simulink model "sschdlexFlybackConverterModel"  (R2026a)
settings: Solver=FixedStepDiscrete  StopTime=200e-6
InitFcn:
  | ts = 2e-008;
libraries: fl_lib x13, nesl_utility x7, ee_lib x2, simulink x1, hdlsllib x1
CloseFcn:
  | clear ts;
settings Model: DataTypeOverride=Off  Creator=The MathWorks, Inc.  LastModifiedBy=The MathWorks, Inc.
settings OptimizationCC: ConditionallyExecuteInputs=off
settings DebuggingCC: AlgebraicLoopMsg=error  SingleTaskRateTransMsg=error  ParameterPrecisionLossMsg=none
settings HardwareCC: ProdHWDeviceType=ASIC/FPGA->ASIC/FPGA  TargetBitPerLong=64.0  TargetBitPerPointer=64.0  TargetBitPerSizeT=64.0  TargetBitPerPtrDiffT=64.0  TargetLongLongMode=on  TargetIntDivRoundTo=Zero  TargetEndianess=LittleEndian  TargetWordSize=64.0  TargetHWDeviceType=Custom Processor->MATLAB Host Computer  ProdEqTarget=off
settings SimscapeCC: SimscapeNominalValues="[{\"value\":\"1\",\"unit\":\"A\"},{\"value\":\"1\",\"unit\":\"bar\"},{\"value\":\"1\",\"unit\":\"cm^2\"},{\"value\":\"1\",\"unit\":\"cm^3/s\"},{\"value\":\"1\",\"unit\":\"kJ/kg\"},{\"value\":\"1\",\"unit\":\"kW\"},{\"value\":\"1\",\"unit\":\"l\"},{\"value\":\"1\",\"unit\":\"N\"},{\"value\":\"1\",\"unit\":\"N*m\"},{\"value\":\"1\",\"unit\":\"V\"}]"  SimscapeLogType=none  SimscapeLogDataHistory=5000.0

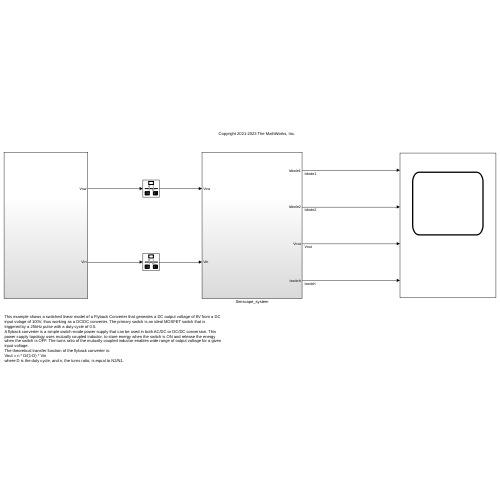
[thumbnail: Simulink's stored preview of the top-level diagram]
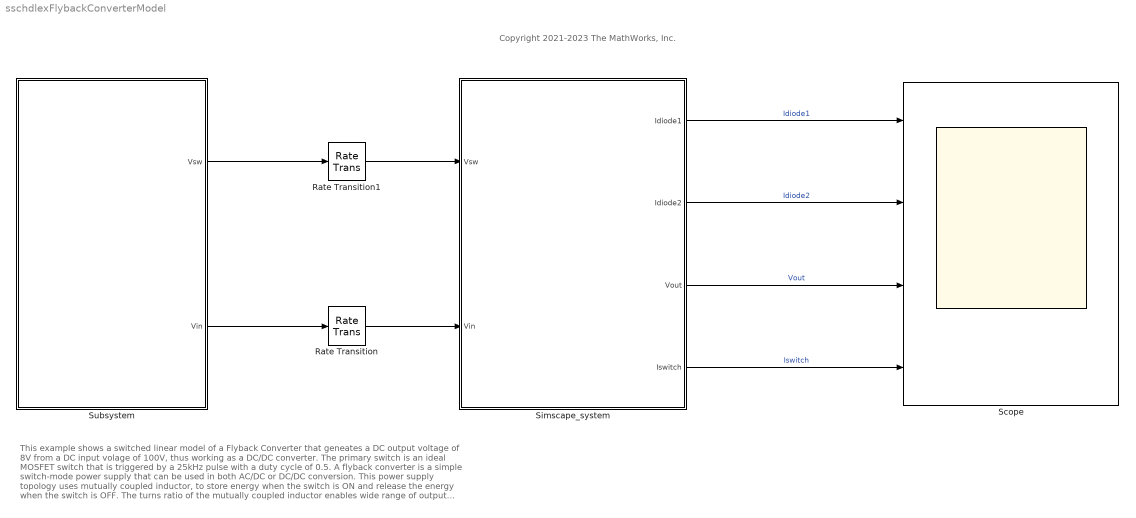
== system sschdlexFlybackConverterModel ==
  note: This example shows a switched linear model of a Flyback Converter that geneates a DC output voltage of 8V from a DC input volage of 100V, thus working as a DC/DC converter. The primary switch is an ideal MOSFET switch that is triggered by a 25kHz pulse with a duty cycle of 0.5.
      | A flyback converter is a simple switch-mode power supply that can be used in both AC/DC or DC/DC conversion. This power supply topology uses mutually coupled inductor, to store energy when the switch is ON and release the energy when the switch is OFF. The turns ratio of the mutually coupled inductor enables wide range of output voltage for a given input voltage.
      | The theoretical transfer function of the flyback converter is:
      | Vout = n * D/(1-D) * Vin
      | where D is the duty cycle, and n, the turns ratio, is equal to N2/N1.
  note: Copyright 2021-2023 The MathWorks, Inc.
  Rate Transition : RateTransition
  Rate Transition1 : RateTransition
  Scope : Scope  NumInputPorts=4
      settings: ActiveDisplayYMinimum=-0.32624  ActiveDisplayYMaximum=2.75944
  Simscape_system : Subsystem
  Subsystem : Subsystem
  wires:
  Subsystem/1(Vsw) -> Rate Transition1/1
  Subsystem/2(Vin) -> Rate Transition/1
  Rate Transition1/1 -> Simscape_system/1(Vsw)
  Rate Transition/1 -> Simscape_system/2(Vin)
  Simscape_system/1(Idiode1) -> Scope/1  "Idiode1"
  Simscape_system/2(Idiode2) -> Scope/2  "Idiode2"
  Simscape_system/3(Vout) -> Scope/3  "Vout"
  Simscape_system/4(Iswitch) -> Scope/4  "Iswitch"

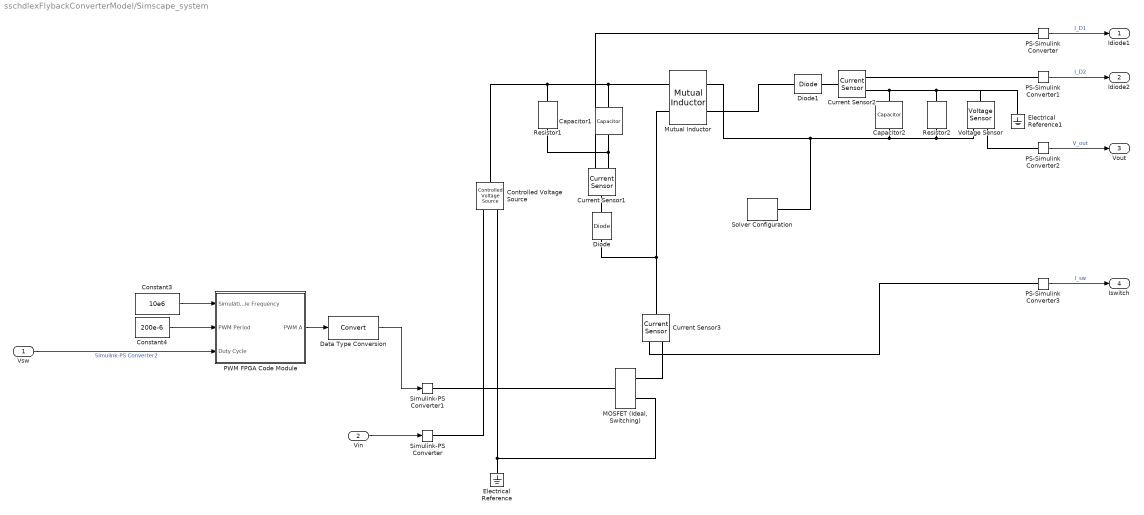
== system sschdlexFlybackConverterModel/Simscape_system ==
  Vsw : Inport
  Vin : Inport  Port=2
  Capacitor1 : fl_lib/Electrical/Electrical Elements/Capacitor  c=0.1e-12 F  r=0 Ohm  g=0 1/Ohm  i_specify=off  i_priority=None  i=0 A  i_nominal_specify=off  i_nominal_value=1  i_nominal_unit=A  v_specify=off  v_priority=None  v=0 V  v_nominal_specify=off  v_nominal_value=1  v_nominal_unit=V  vc_specify=off  vc_priority=High  vc=0 V  vc_nominal_specify=off  vc_nominal_value=1  vc_nominal_unit=V
  Capacitor2 : fl_lib/Electrical/Electrical Elements/Capacitor  c=50e-6 F  r=0 Ohm  g=0 1/Ohm  i_specify=off  i_priority=None  i=0 A  i_nominal_specify=off  i_nominal_value=1  i_nominal_unit=A  v_specify=off  v_priority=None  v=0 V  v_nominal_specify=off  v_nominal_value=1  v_nominal_unit=V  vc_specify=on  vc_priority=High  vc=8 V  vc_nominal_specify=off  vc_nominal_value=1  vc_nominal_unit=V
  Constant3 : Constant  Value=10e6  OutDataTypeStr=single  SampleTime=-1
  Constant4 : Constant  Value=200e-6  OutDataTypeStr=single  SampleTime=-1
  Controlled Voltage Source : fl_lib/Electrical/Electrical Sources/Controlled Voltage Source
  Current Sensor1 : fl_lib/Electrical/Electrical Sensors/Current Sensor
  Current Sensor2 : fl_lib/Electrical/Electrical Sensors/Current Sensor
  Current Sensor3 : fl_lib/Electrical/Electrical Sensors/Current Sensor
  Data Type Conversion : DataTypeConversion  SaturateOnIntegerOverflow=off  RndMeth=Floor
  Diode : fl_lib/Electrical/Electrical Elements/Diode  Vf=0.001 V  Ron=0.001 Ohm  Goff=1e-6 1/Ohm  i_specify=off  i_priority=None  i=0 A  i_nominal_specify=off  i_nominal_value=1  i_nominal_unit=A  v_specify=off  v_priority=None  v=0 V  v_nominal_specify=off  v_nominal_value=1  v_nominal_unit=V
  Diode1 : fl_lib/Electrical/Electrical Elements/Diode  Vf=0.25 V  Ron=0.3 Ohm  Goff=1e-8 1/Ohm  i_specify=off  i_priority=None  i=0 A  i_nominal_specify=off  i_nominal_value=1  i_nominal_unit=A  v_specify=off  v_priority=None  v=0 V  v_nominal_specify=off  v_nominal_value=1  v_nominal_unit=V
  Electrical Reference : fl_lib/Electrical/Electrical Elements/Electrical Reference
  Electrical Reference1 : fl_lib/Electrical/Electrical Elements/Electrical Reference
  "MOSFET (Ideal, Switching)" : ee_lib/Semiconductors & Converters/MOSFET (Ideal, Switching)  port_option=ee.enum.controlport.ps  Rds=1e-9 Ohm  Goff=1e-9 1/Ohm  Vth=0.001 V  diode_param=1  diode_Vf=0.8 V  diode_Ron=0.001 Ohm  diode_Goff=1e-5 1/Ohm  diode_C=50e-9 F  diode_iRM=-235 A  diode_iF=300 A  diode_idot=-50 A/us  diode_trr_param=1  diode_trr_factor=3  diode_trr=15 us  diode_Qrr=1500 s*uA  ids_specify=off  ids_priority=None  ids=0 A  ids_nominal_specify=off  ids_nominal_value=1  ids_nominal_unit=A  vds_specify=off  vds_priority=None  vds=0 V  vds_nominal_specify=off  vds_nominal_value=1  vds_nominal_unit=V  vgs_specify=off  vgs_priority=None  vgs=0 V  vgs_nominal_specify=off  vgs_nominal_value=1  vgs_nominal_unit=V  thermal_loss_option=ee.enum.converters.thermalLossOption.constantvalues  Von_data=[0, 1.8, 3.2, 6, 10, 16; 0, 2, 5.5, 9.5, 15, 25] V  Tj=[298.15, 448.15] K  Iout_data=[0, 20, 40, 60, 80, 100] A  tabulateWithVds=false  Eon_data=[0, 55.04, 124.57, 235.53, 362.12; 0, 71.25, 161.25, 304.88, 468.75] * 1e-6 J  Eoff_data=[0, 18, 30, 56.1, 76.5; 0, 22.5, 37.5, 70.13, 95.63] * 1e-6 J  Eon_data_3D=[zeros(2, 5, 3)] J  Eoff_data_3D=[zeros(2, 5, 3)] J  Tj_loss=[298.15, 448.15] K  Iout_data_loss=[0, 10, 20, 30, 40] A  Vds_loss=[0, 150, 300] V  Eon_scalar=22.86e-3 J  Eoff_scalar=17.14e-3 J  Voff=300 V  Iout_scalar=600 A  useCurrentFromPreviousCycle=false  useVoltageFromPreviousCycle=false  diodeModelType=ee.enum.converters.diodeModelType.pwl  diodeTableType=ee.enum.diode.tableType.IfMat  diode_ReverseIVType=ee.enum.diode.diodeReverseIV.constant  diode_IfMat=[.07, .12, .19, 1.75, 4.24, 7.32, 11.2; .16, .3, .72, 2.14, 4.02, 6.35, 9.12] A  diode_VfMat=[.9, 1.15, 1.25, 1.5, 1.75, 2.17, 2.6, 2.85; .58, .68, .75, 1.1, 1.38, 1.77, 2.27, 2.7] V  diode_TjVec=[25, 125] degC  diode_VfVec=[.5, .7, .9, 1.3, 1.7, 2.1, 2.5] V  diode_IfVec=[.1, .2, .5, 1, 2, 4, 7, 10] A  diode_IrMat=[1e-06, 2e-06, 5e-06, 1e-05, 2.5e-05, 5e-05, .0001; 2e-06, 5e-06, 1e-05, 4e-05, 8e-05, .0002, .0005] A  diode_VrMat=[10, 100, 200, 250, 300, 325, 350; 10, 70, 160, 220, 270, 300, 320] V  diode_VrVec=[10, 20, 40, 50, 70, 80, 100] V  diode_IrVec=[1e-06, 2e-06, 5e-06, 1e-05, 2e-05, 5e-05, .0001] A  diode_Vr=-600 V  diode_Ls=150 nH  diode_Erec=0.03 J  diode_rec_loss_model=ee.enum.diode.reverseRecoveryModel.fixed  diode_ErecVal=0 J  diode_scaleWithIandV=true  diode_ErecMat=zeros(2, 3) J  diodeErecMat3D=zeros(2, 3, 2) J  diode_TjrecVec=[298.15, 398.15] K  diode_IfrecVec=[.1, 1, 10] A  diodeVrecVec=[0, 100] V  diode_IrecVal=10 A  diode_VrecVal=10 V  diode_tFilter=1 / 1000 / 100 s  separateThermalPortForDiode=false  thermal_network_parameterization=ee.enum.thermalNetworkTopology.external  Rth=[.03, .2] K/W  Rth_Cauer=[.03, .1, .2] K/W  Rth_Foster=[.03, .2] K/W  thermal_mass_parameterization=ee.enum.thermalNetwork.timeconstant  thermal_mass=[3, 25] J/K  thermal_mass_Cauer=[3, 10, 25] J/K  thermal_mass_Foster=[33, 50] J/K  thermal_time_constant=[.1, 5] s  thermal_time_constant_Cauer=[.1, 1, 5] s  thermal_time_constant_Foster=[1, 10] s  thermal_mass_initial_temperatures=[25, 25] degC  thermal_mass_initial_temperatures_Cauer=[25, 25, 25] degC  junction_thermal_mass=0.1 J/K  Tvec_initial_Foster=[25, 25, 25, 25] degC  RthDiode=[.03, .2] K/W  RthCauerDiode=[.03, .1, .2] K/W  RthFosterDiode=[.03, .2] K/W  thermalMassDiode=[3, 25] J/K  thermalMassCauerDiode=[3, 10, 25] J/K  thermalMassFosterDiode=[33, 50] J/K  thermalTauDiode=[.1, 5] s  thermalTauCauerDiode=[.1, 1, 5] s  thermalTauFosterDiode=[1, 10] s  thermalMassInitTempDiode=[25, 25] degC  thermalMassInitTempCauerDiode=[25, 25, 25] degC  junctionthermalMassDiode=0.1 J/K  TVecInitialFosterDiode=[25, 25, 25, 25] degC  no_thermal_network=0  mosfet_junction_temperature_specify=off  mosfet_junction_temperature_priority=None  mosfet_junction_temperature=25 degC  mosfet_junction_temperature_nominal_specify=off  mosfet_junction_temperature_nominal_value=1  mosfet_junction_temperature_nominal_unit=degC  diode_junction_temperature_specify=off  diode_junction_temperature_priority=None  diode_junction_temperature=25 degC  diode_junction_temperature_nominal_specify=off  diode_junction_temperature_nominal_value=1  diode_junction_temperature_nominal_unit=degC  Qj_specify=off  Qj_priority=None  Qj=0 W  Qj_nominal_specify=off  Qj_nominal_value=1  Qj_nominal_unit=W  accumulatedSwitchingLosses_specify=off  accumulatedSwitchingLosses_priority=None  accumulatedSwitchingLosses=0 J
  Mutual Inductor : ee_lib/Passive/Transformers/Mutual Inductor  L1=10 uH  L2=10 uH  k=0.08  L_tol=5  enable_L1_tol=0  L1_tol_distribution=1  L1_nSigma=4  enable_L2_tol=0  L2_tol_distribution=1  L2_nSigma=4  r=[.1e-3, .1e-3] Ohm  g=[1e-09, 1e-09] 1/Ohm  enable_operating_limits=0  operating_limit_action=2  max_working_current=1 A  power_rating=1 W  iL1_specify=off  iL1_priority=High  iL1=0 A  iL1_nominal_specify=off  iL1_nominal_value=1  iL1_nominal_unit=A  iL2_specify=off  iL2_priority=High  iL2=0 A  iL2_nominal_specify=off  iL2_nominal_value=1  iL2_nominal_unit=A
  PS-Simulink Converter{,1..3} (4 alike) : nesl_utility/PS-Simulink Converter  PhysicalDomain=network_engine_domain  SubClassName=ps_output  LeftPortType=input  RightPortType=output  PseudoPeriodic=off  Frequencies=[]  VectorFormat=1-D array  Unit=inherit  AffineConversion=off
  PWM FPGA Code Module : Subsystem  SystemSampleTime=1/75e6
  Resistor1 : fl_lib/Electrical/Electrical Elements/Resistor  R=50e3 Ohm  i_specify=off  i_priority=None  i=0 A  i_nominal_specify=off  i_nominal_value=1  i_nominal_unit=A  v_specify=off  v_priority=None  v=0 V  v_nominal_specify=off  v_nominal_value=1  v_nominal_unit=V
  Resistor2 : fl_lib/Electrical/Electrical Elements/Resistor  R=2.5 Ohm  i_specify=off  i_priority=None  i=0 A  i_nominal_specify=off  i_nominal_value=1  i_nominal_unit=A  v_specify=off  v_priority=None  v=0 V  v_nominal_specify=off  v_nominal_value=1  v_nominal_unit=V
  Simulink-PS Converter : nesl_utility/Simulink-PS Converter  PhysicalDomain=network_engine_domain  SubClassName=ps_input  LeftPortType=input  RightPortType=output  PseudoPeriodic=off  Frequencies=[]  NoiseDistribution=none  NoiseParameters=[]  Unit=1  AffineConversion=off  FilteringAndDerivatives=provide  SimscapeFilterOrder=1  InputFilterTimeConstant=0.001  UdotUserProvided=0
  Simulink-PS Converter1 : nesl_utility/Simulink-PS Converter  PhysicalDomain=network_engine_domain  SubClassName=ps_input  LeftPortType=input  RightPortType=output  PseudoPeriodic=off  Frequencies=[]  NoiseDistribution=none  NoiseParameters=[]  Unit=1  AffineConversion=off  FilteringAndDerivatives=provide  SimscapeFilterOrder=1  InputFilterTimeConstant=0.001  UdotUserProvided=0
  Solver Configuration : nesl_utility/Solver Configuration  PhysicalDomain=network_engine_domain  SubClassName=solver  LeftPortType=input  RightPortType=generic  Tones=[]  Harmonics=[]  SimulateNoise=off  Profile=off  UseLocalSampling=off  EnableSwitchedLinearOptims=on  FrequencyDomain=off  UseCCode=off  RelTol=0.001  AbsTol=1e-06  MinStep=1e-09  ToWorkspace=off  RevertToSquareIcSolve=off  NumHomotopyIterations=100  PhasorMode=off  PhasorModeNumHarmonics=1  ConsistencySolver=NEWTON_FTOL  CanonicalOrdering=UNORDERED  OptimizeIntermediates=UNOPTIMIZED  IndexReductionMethod=DerivativeReplacement  DoDC=off  ResidualTolerance=1e-09  ConsistencyTolSource=GLOBAL  ConsistencyAbsTol=0.001  ConsistencyRelTol=0.001  ConsistencyTolFactor=0.001  UseLocalSolver=on  LocalSolverChoice=NE_BACKWARD_EULER_ADVANCER  ResolveIndetEquations=on  FunctionEvalNumThread=1  LocalSolverSampleTime=ts  DoFixedCost=on  MaxNonlinIter=3  MaxModeIter=2  ComputeImpulses=off  ImpulseIterations=1  LinearAlgebra=auto  LinearAlgebraNumThread=0  EquationFormulation=NE_TIME_EF  DelaysMemoryBudget=1024  AutomaticFiltering=on  FilteringTimeConstant=0.001  PartitionStorageMethod=AS_NEEDED  PartitionMemoryBudget=1024  PartitionMethod=ROBUST  MultibodyUseLocalSolver=off  MultibodyLocalSolverChoice=ODE1  MultibodyLocalSolverSampleTime=0.001
  Voltage Sensor : fl_lib/Electrical/Electrical Sensors/Voltage Sensor
  Idiode1 : Outport
  Idiode2 : Outport  Port=2
  Vout : Outport  Port=3
  Iswitch : Outport  Port=4
  wires:
  Data Type Conversion/1 -> Simulink-PS Converter1/1
  Vin/1 -> Simulink-PS Converter/1
  PS-Simulink Converter2/1 -> Vout/1  "V_out"
  PS-Simulink Converter1/1 -> Idiode2/1  "I_D2"
  PS-Simulink Converter/1 -> Idiode1/1  "I_D1"
  PS-Simulink Converter3/1 -> Iswitch/1  "I_sw"
  Vsw/1 -> PWM FPGA Code Module/3(Duty Cycle)  "Simulink-PS Converter2"
  Constant4/1 -> PWM FPGA Code Module/2(PWM Period)
  PWM FPGA Code Module/1(PWM A) -> Data Type Conversion/1
  Constant3/1 -> PWM FPGA Code Module/1(Simulation Sample Frequency)
  connections:
  Diode/RConn1 -- Current Sensor1/LConn1
  Electrical Reference/LConn1 -- "MOSFET (Ideal, Switching)"/RConn2 -- Controlled Voltage Source/RConn2
  "MOSFET (Ideal, Switching)"/LConn1 -- Simulink-PS Converter1/RConn1
  Capacitor1/RConn1 -- Resistor1/RConn1 -- Current Sensor1/RConn2
  Current Sensor3/LConn1 -- Diode/LConn1 -- Mutual Inductor/LConn2
  Current Sensor1/RConn1 -- PS-Simulink Converter/LConn1
  Diode1/RConn1 -- Current Sensor2/LConn1
  PS-Simulink Converter2/LConn1 -- Voltage Sensor/RConn1
  Current Sensor2/RConn2 -- Capacitor2/LConn1 -- Resistor2/LConn1 -- Electrical Reference1/LConn1 -- Voltage Sensor/LConn1
  Simulink-PS Converter/RConn1 -- Controlled Voltage Source/RConn1
  Controlled Voltage Source/LConn1 -- Resistor1/LConn1 -- Mutual Inductor/LConn1 -- Capacitor1/LConn1
  Solver Configuration/RConn1 -- Mutual Inductor/RConn1 -- Capacitor2/RConn1 -- Resistor2/RConn1 -- Voltage Sensor/RConn2
  PS-Simulink Converter1/LConn1 -- Current Sensor2/RConn1
  PS-Simulink Converter3/LConn1 -- Current Sensor3/RConn1
  Current Sensor3/RConn2 -- "MOSFET (Ideal, Switching)"/RConn1
  Diode1/LConn1 -- Mutual Inductor/RConn2

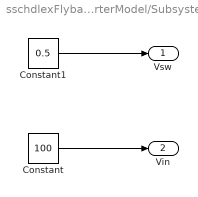
== system sschdlexFlybackConverterModel/Subsystem ==
  Constant : Constant  Value=100  SampleTime=0
  Constant1 : Constant  Value=0.5  SampleTime=ts
  Vsw : Outport
  Vin : Outport  Port=2
  wires:
  Constant1/1 -> Vsw/1
  Constant/1 -> Vin/1

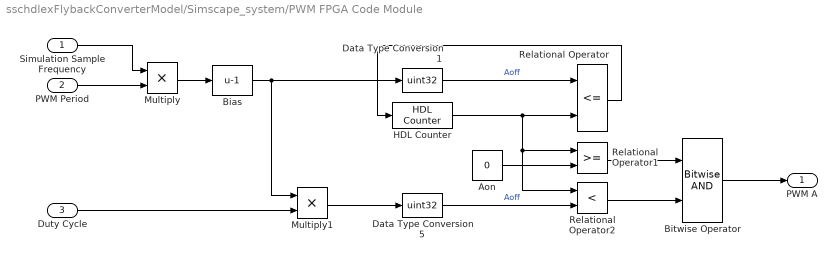
== system sschdlexFlybackConverterModel/Simscape_system/PWM FPGA Code Module ==
  Simulation Sample Frequency : Inport
  PWM Period : Inport  Port=2
  Duty Cycle : Inport  Port=3
  Aon : Constant  Value=0  OutDataTypeStr=uint32  SampleTime=-1
  Bias : Bias  Bias=-1  SaturateOnIntegerOverflow=off
  Bitwise Operator : simulink/Logic and Bit Operations/Bitwise Operator  logicop=AND  UseBitMask=off  NumInputPorts=2  BitMask=bin2dec('11011001')  BitMaskRealWorld=Stored Integer
  Data Type Conversion1 : DataTypeConversion  OutDataTypeStr=uint32  SaturateOnIntegerOverflow=off  RndMeth=Floor
  Data Type Conversion5 : DataTypeConversion  OutDataTypeStr=uint32  SaturateOnIntegerOverflow=off  RndMeth=Floor
  HDL Counter : hdlsllib/Sources/HDL Counter  CountType=Free running  CountInit=0  CountStep=1  CountMax=25  CountFromType=Initial value  CountFrom=0  CountResetPort=on  CountLoadPort=off  CountEnbPort=off  CountDirPort=off  CountHitOutputPort=off  CountDataType=Unsigned  CountWordLen=32  CountFracLen=0  CountSampTime=1
  Multiply : Product
  Multiply1 : Product
  Relational Operator : RelationalOperator  Operator=<=  OutDataTypeStr=boolean  InputSameDT=off
  Relational Operator1 : RelationalOperator  OutDataTypeStr=boolean  InputSameDT=off
  Relational Operator2 : RelationalOperator  Operator=<  OutDataTypeStr=boolean  InputSameDT=off
  PWM A : Outport  VectorParamsAs1DForOutWhenUnconnected=off
  wires:
  Bias/1 -> Data Type Conversion1/1, Multiply1/1
  Relational Operator/1 -> HDL Counter/1
  Aon/1 -> Relational Operator1/2
  Data Type Conversion5/1 -> Relational Operator2/2  "Aoff"
  Relational Operator1/1 -> Bitwise Operator/1
  Relational Operator2/1 -> Bitwise Operator/2
  Bitwise Operator/1 -> PWM A/1
  HDL Counter/1 -> Relational Operator2/1, Relational Operator1/1, Relational Operator/2
  PWM Period/1 -> Multiply/2
  Multiply/1 -> Bias/1
  Multiply1/1 -> Data Type Conversion5/1
  Simulation Sample Frequency/1 -> Multiply/1
  Duty Cycle/1 -> Multiply1/2
  Data Type Conversion1/1 -> Relational Operator/1  "Aoff"
